simulink model "original"  (R2025a)
settings: Solver=VariableStepAuto  StartTime=0.0  StopTime=800  RelTol=1e-3
undefined symbols (not defined in the file): D1, Delta
libraries: spsThreePhaseSeriesRLCBranchLib x20, spsThreePhaseVIMeasurementLib x18, spsThreePhaseSeriesRLCLoadLib x11, spsRMSLib x8, spsThreePhaseSourceLib x5, spsThreePhaseTransformerTwoWindingsLib x5, spsPMUPLLBasedPositiveSequenceLib x4, spsCurrentMeasurementLib x3, spsPower3phInstantaneousLib x1, spspowerguiLib x1
settings Model: Creator=Subhalaxmi Sahoo  LastModifiedBy=Subhalaxmi Sahoo

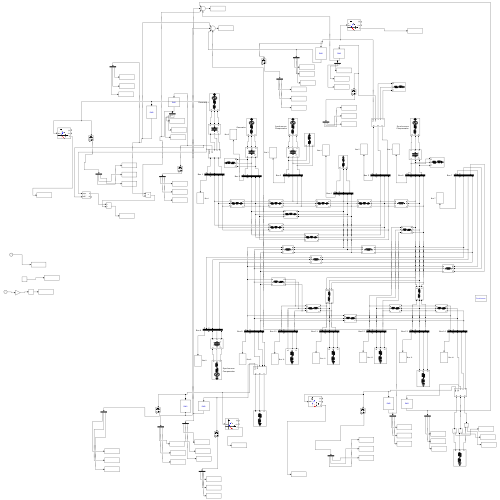
[thumbnail: Simulink's stored preview of the top-level diagram]
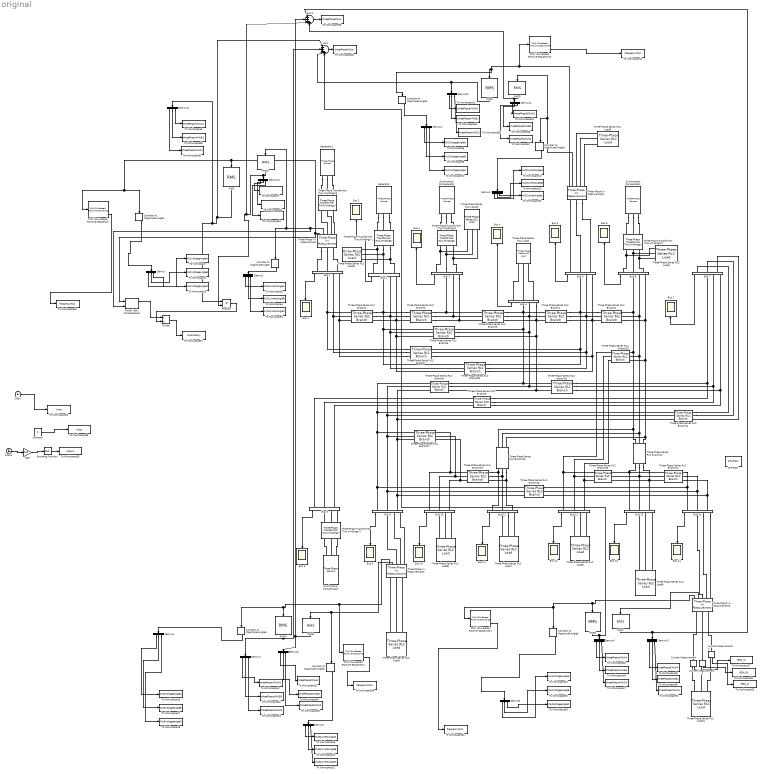
== system original ==
  " Generator" : spsThreePhaseSourceLib/Three-Phase Source  InternalConnection=Yg  VoltagePhases=off  Voltage=1.045  PhaseAngle=-30  Voltage_phases=[25e3 25e3 25e3]/sqrt(3)  PhaseAngles_phases=[0 -120 +120]  Frequency=50  NonIdealSource=on  SpecifyImpedance=on  Resistance=0.8929  Inductance=16.58e-3  ShortCircuitLevel=10  BaseVoltage=1  XRratio=1  BusType=PV  Pref=0.4  Qref=0  Prefabc=[10e3, 10e3, 10e3]  Qrefabc=[0, 0, 0]  Qmin=-0.4  Qmax=0.5
  " Generator1" : spsThreePhaseSourceLib/Three-Phase Source  InternalConnection=Yg  VoltagePhases=off  Voltage=1.06  PhaseAngle=-30  Voltage_phases=[25e3 25e3 25e3]/sqrt(3)  PhaseAngles_phases=[0 -120 +120]  Frequency=50  NonIdealSource=on  SpecifyImpedance=on  Resistance=0.8929  Inductance=16.58e-3  ShortCircuitLevel=10  BaseVoltage=1  XRratio=1  BusType=PQ  Pref=2.324  Qref=-0.169  Prefabc=[10e3, 10e3, 10e3]  Qrefabc=[0, 0, 0]  Qmin=0  Qmax=0
  Bus {1..14} (14 alike) : Scope
      Bus 1 settings: TimeSpan=0.12  ActiveDisplayYMinimum=-1.75  ActiveDisplayYMaximum=1.75
      Bus 10 settings: TimeSpan=0.12  ActiveDisplayYMinimum=-1.5  ActiveDisplayYMaximum=1.5  DataLoggingVariableName=ScopeData9
      Bus 11 settings: TimeSpan=0.12  ActiveDisplayYMinimum=-1.25  ActiveDisplayYMaximum=1.25  DataLoggingVariableName=ScopeData10
      Bus 12 settings: TimeSpan=0.12  ActiveDisplayYMinimum=-1.25  ActiveDisplayYMaximum=1.25  DataLoggingVariableName=ScopeData11
      Bus 13 settings: TimeSpan=0.12  ActiveDisplayYMinimum=-1.25  ActiveDisplayYMaximum=1.25  DataLoggingVariableName=ScopeData12
      Bus 14 settings: TimeSpan=0.12  ActiveDisplayYMinimum=-1.25  ActiveDisplayYMaximum=1.25  DataLoggingVariableName=ScopeData13
      Bus 2 settings: TimeSpan=0.12  ActiveDisplayYMinimum=-1.75  ActiveDisplayYMaximum=1.75
      Bus 3 settings: TimeSpan=0.12  ActiveDisplayYMinimum=-1.75  ActiveDisplayYMaximum=1.75  DataLoggingVariableName=ScopeData6
      Bus 4 settings: TimeSpan=0.12  ActiveDisplayYMinimum=-1.25  ActiveDisplayYMaximum=1.25  DataLoggingVariableName=ScopeData2
      Bus 5 settings: TimeSpan=0.12  ActiveDisplayYMinimum=-1.75  ActiveDisplayYMaximum=2  DataLoggingVariableName=ScopeData3
      Bus 6 settings: TimeSpan=0.12  ActiveDisplayYMinimum=-1.75  ActiveDisplayYMaximum=1.75  DataLoggingVariableName=ScopeData5
      Bus 7 settings: TimeSpan=0.12  ActiveDisplayYMinimum=-1.25  ActiveDisplayYMaximum=1.25  DataLoggingVariableName=ScopeData4
      Bus 8 settings: TimeSpan=0.12  ActiveDisplayYMinimum=-1.1  ActiveDisplayYMaximum=1.1  DataLoggingVariableName=ScopeData7
      Bus 9 settings: TimeSpan=0.12  ActiveDisplayYMinimum=-1  ActiveDisplayYMaximum=0.9  DataLoggingVariableName=ScopeData8
  "Bus 1 " : spsThreePhaseVIMeasurementLib/Three-Phase V-I Measurement  VoltageMeasurement=phase-to-ground  SetLabelV=off  LabelV=Vabc  Vpu=on  VpuLL=off  CurrentMeasurement=yes  SetLabelI=off  LabelI=Iabc  Ipu=on  Pbase=100e6  Vbase=0.95  OutputType=Complex  PhasorSimulation=off  PSBequivalent=0
  "Bus 10 " : spsThreePhaseVIMeasurementLib/Three-Phase V-I Measurement  VoltageMeasurement=phase-to-ground  SetLabelV=off  LabelV=Vabc  Vpu=on  VpuLL=off  CurrentMeasurement=yes  SetLabelI=off  LabelI=Iabc  Ipu=on  Pbase=100e6  Vbase=0.94  OutputType=Complex  PhasorSimulation=off  PSBequivalent=0
  "Bus 11 " : spsThreePhaseVIMeasurementLib/Three-Phase V-I Measurement  VoltageMeasurement=phase-to-ground  SetLabelV=off  LabelV=Vabc  Vpu=on  VpuLL=off  CurrentMeasurement=yes  SetLabelI=off  LabelI=Iabc  Ipu=on  Pbase=100e6  Vbase=0.95  OutputType=Complex  PhasorSimulation=off  PSBequivalent=0
  "Bus 12 " : spsThreePhaseVIMeasurementLib/Three-Phase V-I Measurement  VoltageMeasurement=phase-to-ground  SetLabelV=off  LabelV=Vabc  Vpu=on  VpuLL=off  CurrentMeasurement=yes  SetLabelI=off  LabelI=Iabc  Ipu=on  Pbase=100e6  Vbase=0.95  OutputType=Complex  PhasorSimulation=off  PSBequivalent=0
  "Bus 13 " : spsThreePhaseVIMeasurementLib/Three-Phase V-I Measurement  VoltageMeasurement=phase-to-ground  SetLabelV=off  LabelV=Vabc  Vpu=on  VpuLL=off  CurrentMeasurement=yes  SetLabelI=off  LabelI=Iabc  Ipu=on  Pbase=100e6  Vbase=0.95  OutputType=Complex  PhasorSimulation=off  PSBequivalent=0
  "Bus 14 " : spsThreePhaseVIMeasurementLib/Three-Phase V-I Measurement  VoltageMeasurement=phase-to-ground  SetLabelV=off  LabelV=Vabc  Vpu=on  VpuLL=off  CurrentMeasurement=yes  SetLabelI=off  LabelI=Iabc  Ipu=on  Pbase=100e6  Vbase=0.92  OutputType=Complex  PhasorSimulation=off  PSBequivalent=0
  "Bus 2 " : spsThreePhaseVIMeasurementLib/Three-Phase V-I Measurement  VoltageMeasurement=phase-to-ground  SetLabelV=off  LabelV=Vabc  Vpu=on  VpuLL=off  CurrentMeasurement=yes  SetLabelI=off  LabelI=Iabc  Ipu=on  Pbase=100e6  Vbase=0.95  OutputType=Complex  PhasorSimulation=off  PSBequivalent=0
  "Bus 3 " : spsThreePhaseVIMeasurementLib/Three-Phase V-I Measurement  VoltageMeasurement=phase-to-ground  SetLabelV=off  LabelV=Vabc  Vpu=on  VpuLL=off  CurrentMeasurement=yes  SetLabelI=off  LabelI=Iabc  Ipu=on  Pbase=100e6  Vbase=0.95  OutputType=Complex  PhasorSimulation=off  PSBequivalent=0
  "Bus 4 " : spsThreePhaseVIMeasurementLib/Three-Phase V-I Measurement  VoltageMeasurement=phase-to-ground  SetLabelV=off  LabelV=Vabc  Vpu=on  VpuLL=off  CurrentMeasurement=yes  SetLabelI=off  LabelI=Iabc  Ipu=on  Pbase=100e6  Vbase=0.95  OutputType=Complex  PhasorSimulation=off  PSBequivalent=0
  "Bus 5 " : spsThreePhaseVIMeasurementLib/Three-Phase V-I Measurement  VoltageMeasurement=phase-to-ground  SetLabelV=off  LabelV=Vabc  Vpu=on  VpuLL=off  CurrentMeasurement=yes  SetLabelI=off  LabelI=Iabc  Ipu=on  Pbase=100e6  Vbase=0.95  OutputType=Complex  PhasorSimulation=off  PSBequivalent=0
  "Bus 6 " : spsThreePhaseVIMeasurementLib/Three-Phase V-I Measurement  VoltageMeasurement=phase-to-ground  SetLabelV=off  LabelV=Vabc  Vpu=on  VpuLL=off  CurrentMeasurement=yes  SetLabelI=off  LabelI=Iabc  Ipu=on  Pbase=100e6  Vbase=0.95  OutputType=Complex  PhasorSimulation=off  PSBequivalent=0
  "Bus 7 " : spsThreePhaseVIMeasurementLib/Three-Phase V-I Measurement  VoltageMeasurement=phase-to-ground  SetLabelV=off  LabelV=Vabc  Vpu=on  VpuLL=off  CurrentMeasurement=yes  SetLabelI=off  LabelI=Iabc  Ipu=off  Pbase=100e6  Vbase=0.95  OutputType=Complex  PhasorSimulation=off  PSBequivalent=0
  "Bus 8 " : spsThreePhaseVIMeasurementLib/Three-Phase V-I Measurement  VoltageMeasurement=phase-to-ground  SetLabelV=off  LabelV=Vabc  Vpu=on  VpuLL=off  CurrentMeasurement=yes  SetLabelI=off  LabelI=Iabc  Ipu=on  Pbase=100e6  Vbase=1  OutputType=Complex  PhasorSimulation=off  PSBequivalent=0
  "Bus 9 " : spsThreePhaseVIMeasurementLib/Three-Phase V-I Measurement  VoltageMeasurement=phase-to-ground  SetLabelV=off  LabelV=Vabc  Vpu=on  VpuLL=off  CurrentMeasurement=yes  SetLabelI=off  LabelI=Iabc  Ipu=on  Pbase=100e6  Vbase=0.94  OutputType=Complex  PhasorSimulation=off  PSBequivalent=0
  Clock : Clock
  Clock1 : Clock
  Complex to Magnitude-Angle{,1..6} (7 alike) : ComplexToMagnitudeAngle
  Constant : Constant  Value=0
  Current Measurement : spsCurrentMeasurementLib/Current Measurement  PhasorSimulation=off  OutputType=Complex  PSBequivalent=0
  Current Measurement1 : spsCurrentMeasurementLib/Current Measurement  PhasorSimulation=off  OutputType=Complex  PSBequivalent=0
  Current Measurement2 : spsCurrentMeasurementLib/Current Measurement  PhasorSimulation=off  OutputType=Complex  PSBequivalent=0
  Demux{,1..14} (15 alike) : Demux  Outputs=3
  Divide : Product  Inputs=//
  Gain : Gain  Gain=100
  PMU (PLL-Based, Positive-Sequence){,1..3} (4 alike) : spsPMUPLLBasedPositiveSequenceLib/PMU (PLL-Based, Positive-Sequence)  nominalFrequency=60  samplingRate=64  reportingFactor=1
      settings: LibrarySourceBlock=|
      | sps_lib/Sensors and Measurements/PMU
      | (PLL-Based,
      | Positive-Sequence)
  "Power (3ph, Instantaneous)" : spsPower3phInstantaneousLib/Power (3ph, Instantaneous)
  Product : Product
  RMS{,1..7} (8 alike) : spsRMSLib/RMS  TrueRMS=on  Freq=50  RMSInit=1  Ts=0
  Rounding Function : Rounding
  Sum : Sum  Inputs=|++++
  Sum1 : Sum  Inputs=|++++
  Synchronous Compensator : spsThreePhaseSourceLib/Three-Phase Source  InternalConnection=Yg  VoltagePhases=off  Voltage=1.09  PhaseAngle=-30  Voltage_phases=[25e3 25e3 25e3]/sqrt(3)  PhaseAngles_phases=[0 -120 +120]  Frequency=50  NonIdealSource=on  SpecifyImpedance=on  Resistance=0.8929  Inductance=16.58e-3  ShortCircuitLevel=10  BaseVoltage=1  XRratio=1  BusType=PV  Pref=0  Qref=0  Prefabc=[10e3, 10e3, 10e3]  Qrefabc=[0, 0, 0]  Qmin=-0.06  Qmax=0.24
  Synchronous Compensator : spsThreePhaseSourceLib/Three-Phase Source  InternalConnection=Yg  VoltagePhases=off  Voltage=1.01  PhaseAngle=-30  Voltage_phases=[25e3 25e3 25e3]/sqrt(3)  PhaseAngles_phases=[0 -120 +120]  Frequency=50  NonIdealSource=on  SpecifyImpedance=on  Resistance=0.8929  Inductance=16.58e-3  ShortCircuitLevel=10  BaseVoltage=1  XRratio=1  BusType=PV  Pref=0  Qref=23.4e6  Prefabc=[10e3, 10e3, 10e3]  Qrefabc=[0, 0, 0]  Qmin=0  Qmax=0.4
  "Synchronous Compensator " : spsThreePhaseSourceLib/Three-Phase Source  InternalConnection=Yg  VoltagePhases=off  Voltage=1.07  PhaseAngle=-30  Voltage_phases=[25e3 25e3 25e3]/sqrt(3)  PhaseAngles_phases=[0 -120 +120]  Frequency=50  NonIdealSource=on  SpecifyImpedance=on  Resistance=0.8929  Inductance=16.58e-3  ShortCircuitLevel=10  BaseVoltage=1  XRratio=1  BusType=PV  Pref=0  Qref=23.4e6  Prefabc=[10e3, 10e3, 10e3]  Qrefabc=[0, 0, 0]  Qmin=-0.06  Qmax=0.24
  Three-Phase Series RLC Branch1 : spsThreePhaseSeriesRLCBranchLib/Three-Phase Series RLC Branch  LConnTagsString=A|B|C  RConnTagsString=A|B|C  BranchType=RLC  Resistance=0.01335  Inductance=0.04211/(2*pi*50)  Capacitance=1/0.0128/(2*pi*50)  Measurements=None
  Three-Phase Series RLC Branch10 : spsThreePhaseSeriesRLCBranchLib/Three-Phase Series RLC Branch  LConnTagsString=A|B|C  RConnTagsString=A|B|C  BranchType=L  Resistance=1  Inductance=0.20912/(2*pi*50)  Capacitance=1e-6  Measurements=None
  Three-Phase Series RLC Branch11 : spsThreePhaseSeriesRLCBranchLib/Three-Phase Series RLC Branch  LConnTagsString=A|B|C  RConnTagsString=A|B|C  BranchType=L  Resistance=1  Inductance=0.11001/(2*pi*50)  Capacitance=1e-6  Measurements=None
  Three-Phase Series RLC Branch12 : spsThreePhaseSeriesRLCBranchLib/Three-Phase Series RLC Branch  LConnTagsString=A|B|C  RConnTagsString=A|B|C  BranchType=RL  Resistance=0.06615  Inductance=0.13027/(2*pi*50)  Capacitance=1e-6  Measurements=None
  Three-Phase Series RLC Branch13 : spsThreePhaseSeriesRLCBranchLib/Three-Phase Series RLC Branch  LConnTagsString=A|B|C  RConnTagsString=A|B|C  BranchType=RL  Resistance=0.22092  Inductance=0.19988/(2*pi*50)  Capacitance=1e-6  Measurements=None
  Three-Phase Series RLC Branch14 : spsThreePhaseSeriesRLCBranchLib/Three-Phase Series RLC Branch  LConnTagsString=A|B|C  RConnTagsString=A|B|C  BranchType=RL  Resistance=0.17093  Inductance=0.34802/(2*pi*50)  Capacitance=1e-6  Measurements=None
  Three-Phase Series RLC Branch15 : spsThreePhaseSeriesRLCBranchLib/Three-Phase Series RLC Branch  LConnTagsString=A|B|C  RConnTagsString=A|B|C  BranchType=RL  Resistance=0.12291  Inductance=0.25581/(2*pi*50)  Capacitance=1e-6  Measurements=None
  Three-Phase Series RLC Branch16 : spsThreePhaseSeriesRLCBranchLib/Three-Phase Series RLC Branch  LConnTagsString=A|B|C  RConnTagsString=A|B|C  BranchType=RL  Resistance=0.12711  Inductance=0.27038/(2*pi*50)  Capacitance=1e-6  Measurements=None
  Three-Phase Series RLC Branch17 : spsThreePhaseSeriesRLCBranchLib/Three-Phase Series RLC Branch  LConnTagsString=A|B|C  RConnTagsString=A|B|C  BranchType=RL  Resistance=0.03181  Inductance=0.08450/(2*pi*50)  Capacitance=1e-6  Measurements=None
  Three-Phase Series RLC Branch18 : spsThreePhaseSeriesRLCBranchLib/Three-Phase Series RLC Branch  LConnTagsString=A|B|C  RConnTagsString=A|B|C  BranchType=RL  Resistance=0.09498  Inductance=0.1989/(2*pi*50)  Capacitance=1e-6  Measurements=None
  Three-Phase Series RLC Branch19 : spsThreePhaseSeriesRLCBranchLib/Three-Phase Series RLC Branch  LConnTagsString=A|B|C  RConnTagsString=A|B|C  BranchType=RL  Resistance=0.08205  Inductance=0.19207/(2*pi*50)  Capacitance=1e-6  Measurements=None
  Three-Phase Series RLC Branch2 : spsThreePhaseSeriesRLCBranchLib/Three-Phase Series RLC Branch  LConnTagsString=A|B|C  RConnTagsString=A|B|C  BranchType=RLC  Resistance=0.01938  Inductance=0.05917/(2*pi*50)  Capacitance=1/0.0528/(2*pi*50)  Measurements=None
  Three-Phase Series RLC Branch20 : spsThreePhaseSeriesRLCBranchLib/Three-Phase Series RLC Branch  LConnTagsString=A|B|C  RConnTagsString=A|B|C  BranchType=RLC  Resistance=0.05695  Inductance=0.17388/(2*pi*50)  Capacitance=1/0.0340/(2*pi*50)  Measurements=None
  Three-Phase Series RLC Branch3 : spsThreePhaseSeriesRLCBranchLib/Three-Phase Series RLC Branch  LConnTagsString=A|B|C  RConnTagsString=A|B|C  BranchType=RLC  Resistance=0.04699  Inductance=0.19797/(2*pi*50)  Capacitance=1/0.0438/(2*pi*50)  Measurements=None
  Three-Phase Series RLC Branch4 : spsThreePhaseSeriesRLCBranchLib/Three-Phase Series RLC Branch  LConnTagsString=A|B|C  RConnTagsString=A|B|C  BranchType=L  Resistance=1  Inductance=0.25202/(2*pi*50)  Capacitance=1e-6  Measurements=None
  Three-Phase Series RLC Branch5 : spsThreePhaseSeriesRLCBranchLib/Three-Phase Series RLC Branch  LConnTagsString=A|B|C  RConnTagsString=A|B|C  BranchType=RLC  Resistance=0.06701  Inductance=0.17103/(2*pi*50)  Capacitance=1/0.0346/(2*pi*50)  Measurements=None
  Three-Phase Series RLC Branch6 : spsThreePhaseSeriesRLCBranchLib/Three-Phase Series RLC Branch  LConnTagsString=A|B|C  RConnTagsString=A|B|C  BranchType=RLC  Resistance=0.05811  Inductance=0.17632/(2*pi*50)  Capacitance=1/0.0374/(2*pi*50)  Measurements=None
  Three-Phase Series RLC Branch7 : spsThreePhaseSeriesRLCBranchLib/Three-Phase Series RLC Branch  LConnTagsString=A|B|C  RConnTagsString=A|B|C  BranchType=RLC  Resistance=0.05403  Inductance=0.22304/(2*pi*50)  Capacitance=1/0.0492/(2*pi*50)  Measurements=None
  Three-Phase Series RLC Branch8 : spsThreePhaseSeriesRLCBranchLib/Three-Phase Series RLC Branch  LConnTagsString=A|B|C  RConnTagsString=A|B|C  BranchType=L  Resistance=1  Inductance=0.55618/(2*pi*50)  Capacitance=1e-6  Measurements=None
  Three-Phase Series RLC Branch9 : spsThreePhaseSeriesRLCBranchLib/Three-Phase Series RLC Branch  LConnTagsString=A|B|C  RConnTagsString=A|B|C  BranchType=L  Resistance=1  Inductance=0.17615/(2*pi*50)  Capacitance=1e-6  Measurements=None
  Three-Phase Series RLC Load1 : spsThreePhaseSeriesRLCLoadLib/Three-Phase Series RLC Load  LConnTagsString=A|B|C  Configuration=Y (grounded)  NominalVoltage=1  Vabc=[1e3 1e3 1e3]  Vabcp=[1e3 1e3 1e3]  NominalFrequency=50  UnbalancedPower=off  ActivePower=0.478  InductivePower=0  CapacitivePower=0.039  Pabc=[10e3 9e3 11e3]  QLabc=[100 90 110]  QCabc=[100 90 110]  Pabcp=[10e3 9e3 11e3]  QLabcp=[100 90 110]  QCabcp=[100 90 110]  Measurements=None  LoadType=constant PQ
  Three-Phase Series RLC Load10 : spsThreePhaseSeriesRLCLoadLib/Three-Phase Series RLC Load  LConnTagsString=A|B|C  Configuration=Y (grounded)  NominalVoltage=1  Vabc=[1e3 1e3 1e3]  Vabcp=[1e3 1e3 1e3]  NominalFrequency=50  UnbalancedPower=off  ActivePower=0.149  InductivePower=0.050  CapacitivePower=0  Pabc=[10e3 9e3 11e3]  QLabc=[100 90 110]  QCabc=[100 90 110]  Pabcp=[10e3 9e3 11e3]  QLabcp=[100 90 110]  QCabcp=[100 90 110]  Measurements=None  LoadType=constant Z
  Three-Phase Series RLC Load11 : spsThreePhaseSeriesRLCLoadLib/Three-Phase Series RLC Load  LConnTagsString=A|B|C  Configuration=Y (grounded)  NominalVoltage=1  Vabc=[1e3 1e3 1e3]  Vabcp=[1e3 1e3 1e3]  NominalFrequency=50  UnbalancedPower=off  ActivePower=0.217  InductivePower=0.127  CapacitivePower=0  Pabc=[10e3 9e3 11e3]  QLabc=[100 90 110]  QCabc=[100 90 110]  Pabcp=[10e3 9e3 11e3]  QLabcp=[100 90 110]  QCabcp=[100 90 110]  Measurements=None  LoadType=constant PQ
  Three-Phase Series RLC Load12 : spsThreePhaseSeriesRLCLoadLib/Three-Phase Series RLC Load  LConnTagsString=A|B|C  Configuration=Y (grounded)  NominalVoltage=1  Vabc=[1e3 1e3 1e3]  Vabcp=[1e3 1e3 1e3]  NominalFrequency=50  UnbalancedPower=off  ActivePower=0.942  InductivePower=0.191  CapacitivePower=0  Pabc=[10e3 9e3 11e3]  QLabc=[100 90 110]  QCabc=[100 90 110]  Pabcp=[10e3 9e3 11e3]  QLabcp=[100 90 110]  QCabcp=[100 90 110]  Measurements=None  LoadType=constant PQ
  Three-Phase Series RLC Load3 : spsThreePhaseSeriesRLCLoadLib/Three-Phase Series RLC Load  LConnTagsString=A|B|C  Configuration=Y (grounded)  NominalVoltage=1  Vabc=[1e3 1e3 1e3]  Vabcp=[1e3 1e3 1e3]  NominalFrequency=50  UnbalancedPower=off  ActivePower=0.076  InductivePower=0.016  CapacitivePower=0  Pabc=[10e3 9e3 11e3]  QLabc=[100 90 110]  QCabc=[100 90 110]  Pabcp=[10e3 9e3 11e3]  QLabcp=[100 90 110]  QCabcp=[100 90 110]  Measurements=None  LoadType=constant PQ
  Three-Phase Series RLC Load4 : spsThreePhaseSeriesRLCLoadLib/Three-Phase Series RLC Load  LConnTagsString=A|B|C  Configuration=Y (grounded)  NominalVoltage=1  Vabc=[1e3 1e3 1e3]  Vabcp=[1e3 1e3 1e3]  NominalFrequency=50  UnbalancedPower=off  ActivePower=0.112  InductivePower=0.075  CapacitivePower=0  Pabc=[10e3 9e3 11e3]  QLabc=[100 90 110]  QCabc=[100 90 110]  Pabcp=[10e3 9e3 11e3]  QLabcp=[100 90 110]  QCabcp=[100 90 110]  Measurements=None  LoadType=constant PQ
  Three-Phase Series RLC Load5 : spsThreePhaseSeriesRLCLoadLib/Three-Phase Series RLC Load  LConnTagsString=A|B|C  Configuration=Y (grounded)  NominalVoltage=1  Vabc=[1e3 1e3 1e3]  Vabcp=[1e3 1e3 1e3]  NominalFrequency=50  UnbalancedPower=off  ActivePower=0.295  InductivePower=0.166  CapacitivePower=0  Pabc=[10e3 9e3 11e3]  QLabc=[100 90 110]  QCabc=[100 90 110]  Pabcp=[10e3 9e3 11e3]  QLabcp=[100 90 110]  QCabcp=[100 90 110]  Measurements=None  LoadType=constant PQ
  Three-Phase Series RLC Load6 : spsThreePhaseSeriesRLCLoadLib/Three-Phase Series RLC Load  LConnTagsString=A|B|C  Configuration=Y (grounded)  NominalVoltage=1  Vabc=[1e3 1e3 1e3]  Vabcp=[1e3 1e3 1e3]  NominalFrequency=50  UnbalancedPower=off  ActivePower=0.09  InductivePower=0.058  CapacitivePower=0  Pabc=[10e3 9e3 11e3]  QLabc=[100 90 110]  QCabc=[100 90 110]  Pabcp=[10e3 9e3 11e3]  QLabcp=[100 90 110]  QCabcp=[100 90 110]  Measurements=None  LoadType=constant PQ
  Three-Phase Series RLC Load7 : spsThreePhaseSeriesRLCLoadLib/Three-Phase Series RLC Load  LConnTagsString=A|B|C  Configuration=Y (grounded)  NominalVoltage=1  Vabc=[1e3 1e3 1e3]  Vabcp=[1e3 1e3 1e3]  NominalFrequency=50  UnbalancedPower=off  ActivePower=0.035  InductivePower=0.018  CapacitivePower=0  Pabc=[10e3 9e3 11e3]  QLabc=[100 90 110]  QCabc=[100 90 110]  Pabcp=[10e3 9e3 11e3]  QLabcp=[100 90 110]  QCabcp=[100 90 110]  Measurements=None  LoadType=constant PQ
  Three-Phase Series RLC Load8 : spsThreePhaseSeriesRLCLoadLib/Three-Phase Series RLC Load  LConnTagsString=A|B|C  Configuration=Y (grounded)  NominalVoltage=1  Vabc=[1e3 1e3 1e3]  Vabcp=[1e3 1e3 1e3]  NominalFrequency=50  UnbalancedPower=off  ActivePower=0.061  InductivePower=0.016  CapacitivePower=0  Pabc=[10e3 9e3 11e3]  QLabc=[100 90 110]  QCabc=[100 90 110]  Pabcp=[10e3 9e3 11e3]  QLabcp=[100 90 110]  QCabcp=[100 90 110]  Measurements=None  LoadType=constant PQ
  Three-Phase Series RLC Load9 : spsThreePhaseSeriesRLCLoadLib/Three-Phase Series RLC Load  LConnTagsString=A|B|C  Configuration=Y (grounded)  NominalVoltage=1  Vabc=[1e3 1e3 1e3]  Vabcp=[1e3 1e3 1e3]  NominalFrequency=50  UnbalancedPower=off  ActivePower=0.135  InductivePower=0.058  CapacitivePower=0  Pabc=[10e3 9e3 11e3]  QLabc=[100 90 110]  QCabc=[100 90 110]  Pabcp=[10e3 9e3 11e3]  QLabcp=[100 90 110]  QCabcp=[100 90 110]  Measurements=None  LoadType=constant PQ
  Three-Phase Transformer (Two Windings)1 : spsThreePhaseTransformerTwoWindingsLib/Three-Phase Transformer (Two Windings)  Winding1Connection=Delta (D1)  Winding2Connection=Yg  CoreType=Three single-phase transformers  SetSaturation=off  Hysteresis=off  DataFile='hysteresis'  SetInitialFlux=off  Measurements=None  UNITS=pu  NominalPower=[ 1 , 50 ]  Winding1=[ 1.045 , 0.002 , 0.08 ]  Winding2=[ 1.045 , 0.002 , 0.08 ]  Rm=500  Lm=500  L0=0.5  Saturation=[ 0,0 ; 0.0024,1.2 ; 1.0,1.52 ]  InitialFluxes=[ 0.8 , -0.8 , 0.7 ]  BreakLoop=off  DiscreteSolver=Trapezoidal iterative  DataType=off  TransfoNumber=1
  Three-Phase Transformer (Two Windings)2 : spsThreePhaseTransformerTwoWindingsLib/Three-Phase Transformer (Two Windings)  Winding1Connection=Delta (D1)  Winding2Connection=Yg  CoreType=Three single-phase transformers  SetSaturation=off  Hysteresis=off  DataFile='hysteresis'  SetInitialFlux=off  Measurements=None  UNITS=pu  NominalPower=[ 1 , 50 ]  Winding1=[ 1.01 , 0.002 , 0.08 ]  Winding2=[ 1.01 , 0.002 , 0.08 ]  Rm=500  Lm=500  L0=0.5  Saturation=[ 0,0 ; 0.0024,1.2 ; 1.0,1.52 ]  InitialFluxes=[ 0.8 , -0.8 , 0.7 ]  BreakLoop=off  DiscreteSolver=Trapezoidal iterative  DataType=off  TransfoNumber=1
  Three-Phase Transformer (Two Windings)3 : spsThreePhaseTransformerTwoWindingsLib/Three-Phase Transformer (Two Windings)  Winding1Connection=Delta (D1)  Winding2Connection=Yg  CoreType=Three single-phase transformers  SetSaturation=off  Hysteresis=off  DataFile='hysteresis'  SetInitialFlux=off  Measurements=None  UNITS=pu  NominalPower=[ 1 , 50 ]  Winding1=[ 1.07 , 0.002 , 0.08 ]  Winding2=[ 1.07 , 0.002 , 0.08 ]  Rm=500  Lm=500  L0=0.5  Saturation=[ 0,0 ; 0.0024,1.2 ; 1.0,1.52 ]  InitialFluxes=[ 0.8 , -0.8 , 0.7 ]  BreakLoop=off  DiscreteSolver=Trapezoidal iterative  DataType=off  TransfoNumber=1
  Three-Phase Transformer (Two Windings)4 : spsThreePhaseTransformerTwoWindingsLib/Three-Phase Transformer (Two Windings)  Winding1Connection=Yg  Winding2Connection=Delta (D1)  CoreType=Three single-phase transformers  SetSaturation=off  Hysteresis=off  DataFile='hysteresis'  SetInitialFlux=off  Measurements=None  UNITS=pu  NominalPower=[ 1 , 50 ]  Winding1=[ 1.09 , 0.002 , 0.08]  Winding2=[1.09 , 0.002 , 0.08]  Rm=500  Lm=500  L0=0.5  Saturation=[0 0;0.0023999 1.2;1 1.52]  InitialFluxes=[0.80002 -0.80002 0.69999]  BreakLoop=off  DiscreteSolver=Trapezoidal iterative  DataType=off  TransfoNumber=1
  Three-Phase Transformer (Two Windings)5 : spsThreePhaseTransformerTwoWindingsLib/Three-Phase Transformer (Two Windings)  Winding1Connection=Delta (D1)  Winding2Connection=Yg  CoreType=Three single-phase transformers  SetSaturation=off  Hysteresis=off  DataFile='hysteresis'  SetInitialFlux=off  Measurements=None  UNITS=pu  NominalPower=[ 1 , 50 ]  Winding1=[ 1.06 , 0.002 , 0.08 ]  Winding2=[ 1.06 , 0.002 , 0.08 ]  Rm=500  Lm=500  L0=0.5  Saturation=[ 0,0 ; 0.0024,1.2 ; 1.0,1.52 ]  InitialFluxes=[ 0.8 , -0.8 , 0.7 ]  BreakLoop=off  DiscreteSolver=Trapezoidal iterative  DataType=off  TransfoNumber=1
  Three-Phase V-I Measurement{,1..3} (4 alike) : spsThreePhaseVIMeasurementLib/Three-Phase V-I Measurement  VoltageMeasurement=phase-to-ground  SetLabelV=off  LabelV=Vabc  Vpu=off  VpuLL=off  CurrentMeasurement=yes  SetLabelI=off  LabelI=Iabc  Ipu=off  Pbase=100e6  Vbase=500e3  OutputType=Complex  PhasorSimulation=off  PSBequivalent=0
  To Workspace : ToWorkspace  VariableName=MU1VoltageAngleA  SampleTime=0.2
      settings: Save2DSignal=2-D array (concatenate along first dimension)
  To Workspace1 : ToWorkspace  VariableName=MU1VoltageAngleB  SampleTime=0.2
      settings: Save2DSignal=2-D array (concatenate along first dimension)
  To Workspace10 : ToWorkspace  VariableName=MU2VoltageAngleC  SampleTime=0.2
      settings: Save2DSignal=2-D array (concatenate along first dimension)
  To Workspace11 : ToWorkspace  VariableName=MU2CurrentAngleA  SampleTime=0.2
      settings: Save2DSignal=2-D array (concatenate along first dimension)
  To Workspace12 : ToWorkspace  VariableName=MU2CurrentAngleB  SampleTime=0.2
      settings: Save2DSignal=2-D array (concatenate along first dimension)
  To Workspace13 : ToWorkspace  VariableName=MU2CurrentAngleC  SampleTime=0.2
      settings: Save2DSignal=2-D array (concatenate along first dimension)
  To Workspace14 : ToWorkspace  VariableName=threePhaseVMUA2  SampleTime=0.2
      settings: Save2DSignal=2-D array (concatenate along first dimension)
  To Workspace15 : ToWorkspace  VariableName=threePhaseCMUA2  SampleTime=0.2
      settings: Save2DSignal=2-D array (concatenate along first dimension)
  To Workspace16 : ToWorkspace  VariableName=MU3VoltageAngleA  SampleTime=0.2
      settings: Save2DSignal=2-D array (concatenate along first dimension)
  To Workspace17 : ToWorkspace  VariableName=MU3VoltageAngleB  SampleTime=0.2
      settings: Save2DSignal=2-D array (concatenate along first dimension)
  To Workspace18 : ToWorkspace  VariableName=MU3VoltageAngleC  SampleTime=0.2
      settings: Save2DSignal=2-D array (concatenate along first dimension)
  To Workspace19 : ToWorkspace  VariableName=MU3CurrentAngleA  SampleTime=0.2
      settings: Save2DSignal=2-D array (concatenate along first dimension)
  To Workspace2 : ToWorkspace  VariableName=MU1VoltageAngleC  SampleTime=0.2
      settings: Save2DSignal=2-D array (concatenate along first dimension)
  To Workspace20 : ToWorkspace  VariableName=MU3CurrentAngleB  SampleTime=0.2
      settings: Save2DSignal=2-D array (concatenate along first dimension)
  To Workspace21 : ToWorkspace  VariableName=MU3CurrentAngleC  SampleTime=0.2
      settings: Save2DSignal=2-D array (concatenate along first dimension)
  To Workspace22 : ToWorkspace  VariableName=threePhaseVMUB3  SampleTime=0.2
      settings: Save2DSignal=2-D array (concatenate along first dimension)
  To Workspace23 : ToWorkspace  VariableName=threePhaseCMUA3  SampleTime=0.2
      settings: Save2DSignal=2-D array (concatenate along first dimension)
  To Workspace24 : ToWorkspace  VariableName=MU4VoltageAngleA  SampleTime=0.2
      settings: Save2DSignal=2-D array (concatenate along first dimension)
  To Workspace25 : ToWorkspace  VariableName=MU4VoltageAngleB  SampleTime=0.2
      settings: Save2DSignal=2-D array (concatenate along first dimension)
  To Workspace26 : ToWorkspace  VariableName=MU4VoltageAngleC  SampleTime=0.2
      settings: Save2DSignal=2-D array (concatenate along first dimension)
  To Workspace27 : ToWorkspace  VariableName=IED4_iA  SampleTime=0.2
      settings: Save2DSignal=2-D array (concatenate along first dimension)
  To Workspace28 : ToWorkspace  VariableName=IED4_iB  SampleTime=0.2
      settings: Save2DSignal=2-D array (concatenate along first dimension)
  To Workspace29 : ToWorkspace  VariableName=IED4_iC  SampleTime=0.2
      settings: Save2DSignal=2-D array (concatenate along first dimension)
  To Workspace3 : ToWorkspace  VariableName=MU1CurrentAngleA  SampleTime=0.2
      settings: Save2DSignal=2-D array (concatenate along first dimension)
  To Workspace30 : ToWorkspace  VariableName=threePhaseVMUA4  SampleTime=0.2
      settings: Save2DSignal=2-D array (concatenate along first dimension)
  To Workspace31 : ToWorkspace  VariableName=threePhaseCMUC4  SampleTime=0.2
      settings: Save2DSignal=2-D array (concatenate along first dimension)
  To Workspace32 : ToWorkspace  VariableName=time  SampleTime=0.2
      settings: Save2DSignal=2-D array (concatenate along first dimension)
  To Workspace33 : ToWorkspace  VariableName=sqNum  SampleTime=0.2
      settings: Save2DSignal=2-D array (concatenate along first dimension)
  To Workspace34 : ToWorkspace  VariableName=frequencyMU1  SampleTime=0.2
      settings: Save2DSignal=2-D array (concatenate along first dimension)
  To Workspace35 : ToWorkspace  VariableName=threePhaseVSum  SampleTime=0.2
      settings: Save2DSignal=2-D array (concatenate along first dimension)
  To Workspace36 : ToWorkspace  VariableName=threePhaseCSum  SampleTime=0.2
      settings: Save2DSignal=2-D array (concatenate along first dimension)
  To Workspace37 : ToWorkspace  VariableName=consistency  SampleTime=0.2
      settings: Save2DSignal=2-D array (concatenate along first dimension)
  To Workspace38 : ToWorkspace  VariableName=class  SampleTime=0.2
      settings: Save2DSignal=2-D array (concatenate along first dimension)
  To Workspace39 : ToWorkspace  VariableName=frequencyMU3  SampleTime=0.2
      settings: Save2DSignal=2-D array (concatenate along first dimension)
  To Workspace4 : ToWorkspace  VariableName=MU1CurrentAngleB  SampleTime=0.2
      settings: Save2DSignal=2-D array (concatenate along first dimension)
  To Workspace40 : ToWorkspace  VariableName=frequencyMU4  SampleTime=0.2
      settings: Save2DSignal=2-D array (concatenate along first dimension)
  To Workspace41 : ToWorkspace  VariableName=frequencyMU2  SampleTime=0.2
      settings: Save2DSignal=2-D array (concatenate along first dimension)
  To Workspace42 : ToWorkspace  VariableName=threePhaseVMUA3  SampleTime=0.2
      settings: Save2DSignal=2-D array (concatenate along first dimension)
  To Workspace43 : ToWorkspace  VariableName=threePhaseVMUC3  SampleTime=0.2
      settings: Save2DSignal=2-D array (concatenate along first dimension)
  To Workspace44 : ToWorkspace  VariableName=threePhaseCMUB3  SampleTime=0.2
      settings: Save2DSignal=2-D array (concatenate along first dimension)
  To Workspace45 : ToWorkspace  VariableName=threePhaseCMUC3  SampleTime=0.2
      settings: Save2DSignal=2-D array (concatenate along first dimension)
  To Workspace46 : ToWorkspace  VariableName=threePhaseVMUB4  SampleTime=0.2
      settings: Save2DSignal=2-D array (concatenate along first dimension)
  To Workspace47 : ToWorkspace  VariableName=threePhaseVMUC4  SampleTime=0.2
      settings: Save2DSignal=2-D array (concatenate along first dimension)
  To Workspace48 : ToWorkspace  VariableName=threePhaseCMUB4  SampleTime=0.2
      settings: Save2DSignal=2-D array (concatenate along first dimension)
  To Workspace49 : ToWorkspace  VariableName=threePhaseCMUA4  SampleTime=0.2
      settings: Save2DSignal=2-D array (concatenate along first dimension)
  To Workspace5 : ToWorkspace  VariableName=MU1CurrentAngleC  SampleTime=0.2
      settings: Save2DSignal=2-D array (concatenate along first dimension)
  To Workspace50 : ToWorkspace  VariableName=threePhaseVMUB1  SampleTime=0.2
      settings: Save2DSignal=2-D array (concatenate along first dimension)
  To Workspace51 : ToWorkspace  VariableName=threePhaseVMUC1  SampleTime=0.2
      settings: Save2DSignal=2-D array (concatenate along first dimension)
  To Workspace52 : ToWorkspace  VariableName=threePhaseCurrentMUB1  SampleTime=0.2
      settings: Save2DSignal=2-D array (concatenate along first dimension)
  To Workspace53 : ToWorkspace  VariableName=threePhaseCurrentMUC1  SampleTime=0.2
      settings: Save2DSignal=2-D array (concatenate along first dimension)
  To Workspace54 : ToWorkspace  VariableName=threePhaseVMUB2  SampleTime=0.2
      settings: Save2DSignal=2-D array (concatenate along first dimension)
  To Workspace55 : ToWorkspace  VariableName=threePhaseVMUC2  SampleTime=0.2
      settings: Save2DSignal=2-D array (concatenate along first dimension)
  To Workspace56 : ToWorkspace  VariableName=threePhaseCMUB2  SampleTime=0.2
      settings: Save2DSignal=2-D array (concatenate along first dimension)
  To Workspace57 : ToWorkspace  VariableName=threePhaseCMUC2  SampleTime=0.2
      settings: Save2DSignal=2-D array (concatenate along first dimension)
  To Workspace6 : ToWorkspace  VariableName=threePhaseVMUA1  SampleTime=0.2
      settings: Save2DSignal=2-D array (concatenate along first dimension)
  To Workspace7 : ToWorkspace  VariableName=threePhaseCurrentMUA1  SampleTime=0.2
      settings: Save2DSignal=2-D array (concatenate along first dimension)
  To Workspace8 : ToWorkspace  VariableName=MU2VoltageAngleA  SampleTime=0.2
      settings: Save2DSignal=2-D array (concatenate along first dimension)
  To Workspace9 : ToWorkspace  VariableName=MU2VoltageAngleB  SampleTime=0.2
      settings: Save2DSignal=2-D array (concatenate along first dimension)
  powergui : spspowerguiLib/powergui  Priority=1  SimulationMode=Continuous  SampleTime=50e-6  frequency=60  Iterations=50  frequencyindice=50  Pbase=100e6  ErrMax=1e-4  UnitsV=kV  UnitsW=MW  buscounter=0  FunctionMessages=off  echomessages=off  EnableUseOfTLC=off  CurrentSourceSwitches=on  DisableSnubberDevices=off  DisableRonSwitches=off  DisableVfSwitches=off  DisplayEquations=off  AutomaticDiscreteSolvers=off  SolverType=Tustin  Interpol=off  ExternalGateDelay=off  methode=off  Ts=100  x0status=blocks  SPID=off  SwTol=0  HookPort=off  NonlinearTolerance=1e-4  nMaxIteration=100  ContinueOnMaxIteration=off  RestoreLinks=warning  ResistiveCurrentMeasurement=off  Frange=[0:2:500]  Ylog=off  Xlog=on  ShowGrid=off  save=off  variable=ZData  structure=0  ZoomFFT=off  StartTime=0.0  cycles=1  DisplayStyle=1  fundamental=60  FreqAxis=off  MaxFrequency=1000  frequencyindicesteady=1  RmsSteady=1  display=off
  wires:
  RMS7/1 -> Demux10/1, Sum1/1
  Demux5/2 -> To Workspace20/1
  Demux10/3 -> To Workspace31/1
  Demux3/1 -> To Workspace11/1
  "Power (3ph, Instantaneous)"/1 -> Divide/1
  Clock1/1 -> Gain/1
  "Bus 11 "/1 -> Bus 11/1
  Demux4/3 -> To Workspace18/1
  Demux6/2 -> To Workspace25/1
  "Bus 10 "/1 -> Bus 10/1
  "Bus 13 "/1 -> Bus 13/1
  Demux/3 -> To Workspace2/1
  Complex to Magnitude-Angle/2 -> Demux1/1
  Sum/1 -> To Workspace35/1
  Demux10/2 -> To Workspace48/1
  Three-Phase V-I Measurement2/1 -> "PMU (PLL-Based, Positive-Sequence)1"/1, Complex to Magnitude-Angle4/1, RMS4/1
  Three-Phase V-I Measurement3/2 -> RMS7/1
  Demux11/3 -> To Workspace6/1
  RMS2/1 -> Sum/3, Demux13/1
  Clock/1 -> To Workspace32/1
  Current Measurement/1 -> To Workspace27/1
  RMS3/1 -> Demux14/1, Sum1/4
  Demux1/3 -> To Workspace5/1
  Demux7/3 -> To Workspace43/1
  "Bus 5 "/1 -> Bus 5/1
  Complex to Magnitude-Angle3/2 -> Demux3/1
  Three-Phase V-I Measurement1/1 -> "PMU (PLL-Based, Positive-Sequence)3"/1, Complex to Magnitude-Angle2/1, RMS2/1
  Demux14/3 -> To Workspace57/1
  Demux14/1 -> To Workspace15/1
  "Bus 9 "/1 -> Bus 9/1
  Complex to Magnitude-Angle6/2 -> Demux6/1
  Demux1/1 -> To Workspace3/1
  Demux4/1 -> To Workspace16/1
  "PMU (PLL-Based, Positive-Sequence)"/3 -> To Workspace34/1
  "Bus 12 "/1 -> Bus 12/1
  Demux3/3 -> To Workspace13/1
  Demux5/1 -> To Workspace19/1
  Gain/1 -> Rounding Function/1
  "Bus 2 "/1 -> Bus 2/1
  "Bus 6 "/1 -> Bus 6/1
  Demux13/1 -> To Workspace14/1
  Complex to Magnitude-Angle5/2 -> Demux5/1
  Complex to Magnitude-Angle4/2 -> Demux4/1
  Demux/1 -> To Workspace/1
  Three-Phase V-I Measurement1/2 -> Complex to Magnitude-Angle3/1, RMS3/1
  Demux7/2 -> To Workspace22/1
  Demux11/1 -> To Workspace51/1
  Complex to Magnitude-Angle1/2 -> Demux/1
  "Bus 14 "/1 -> Bus 14/1
  Demux2/2 -> To Workspace9/1
  Product/1 -> Divide/2
  Demux13/2 -> To Workspace54/1
  Current Measurement1/1 -> To Workspace28/1
  Rounding Function/1 -> To Workspace33/1
  Sum1/1 -> To Workspace36/1
  Complex to Magnitude-Angle2/2 -> Demux2/1
  Demux3/2 -> To Workspace12/1
  Three-Phase V-I Measurement/2 -> "Power (3ph, Instantaneous)"/2, Complex to Magnitude-Angle/1, RMS1/1
  Demux11/2 -> To Workspace50/1
  Demux10/1 -> To Workspace49/1
  Demux/2 -> To Workspace1/1
  Demux2/3 -> To Workspace10/1
  Constant/1 -> To Workspace38/1
  Demux14/2 -> To Workspace56/1
  RMS4/1 -> Demux7/1, Sum/2
  "Bus 7 "/1 -> Bus 7/1
  "PMU (PLL-Based, Positive-Sequence)3"/3 -> To Workspace41/1
  Demux2/1 -> To Workspace8/1
  Demux1/2 -> To Workspace4/1
  "PMU (PLL-Based, Positive-Sequence)1"/3 -> To Workspace39/1
  Demux9/3 -> To Workspace47/1
  Three-Phase V-I Measurement/1 -> RMS/1, Complex to Magnitude-Angle1/1, "PMU (PLL-Based, Positive-Sequence)"/1, "Power (3ph, Instantaneous)"/1
  Demux12/1 -> To Workspace7/1
  Demux6/3 -> To Workspace26/1
  Three-Phase V-I Measurement2/2 -> Complex to Magnitude-Angle5/1, RMS5/1
  Demux5/3 -> To Workspace21/1
  "Bus 3 "/1 -> Bus 3/1
  Demux6/1 -> To Workspace24/1
  RMS5/1 -> Demux8/1, Sum1/2
  Demux9/2 -> To Workspace46/1
  Demux8/3 -> To Workspace45/1
  "Bus 8 "/1 -> Bus 8/1
  Demux8/1 -> To Workspace23/1
  Demux7/1 -> To Workspace42/1
  "Bus 4 "/1 -> Bus 4/1
  RMS/1 -> Product/1, Demux11/1, Sum/1
  Demux4/2 -> To Workspace17/1
  "PMU (PLL-Based, Positive-Sequence)2"/3 -> To Workspace40/1
  Current Measurement2/1 -> To Workspace29/1
  Divide/1 -> To Workspace37/1
  Demux8/2 -> To Workspace44/1
  Three-Phase V-I Measurement3/1 -> "PMU (PLL-Based, Positive-Sequence)2"/1, Complex to Magnitude-Angle6/1, RMS6/1
  Demux13/3 -> To Workspace55/1
  Demux12/2 -> To Workspace52/1
  Demux9/1 -> To Workspace30/1
  "Bus 1 "/1 -> Bus 1/1
  RMS6/1 -> Demux9/1, Sum/4
  RMS1/1 -> Demux12/1, Sum1/3, Product/2
  Demux12/3 -> To Workspace53/1
  connections:
  Three-Phase Series RLC Branch7/LConn3 -- "Bus 1 "/RConn3 -- Three-Phase Series RLC Branch2/LConn3
  Three-Phase Series RLC Branch3/RConn2 -- "Bus 3 "/RConn2 -- Three-Phase Series RLC Branch5/LConn2
  Three-Phase Series RLC Branch7/LConn2 -- "Bus 1 "/RConn2 -- Three-Phase Series RLC Branch2/LConn2
  Three-Phase Transformer (Two Windings)3/RConn3 -- "Bus 6 "/LConn3 -- Three-Phase Series RLC Load4/LConn3
  Three-Phase Series RLC Branch3/LConn1 -- "Bus 2 "/RConn1 -- Three-Phase Series RLC Branch20/LConn1 -- Three-Phase Series RLC Branch6/LConn1 -- Three-Phase Series RLC Branch2/RConn1
  Three-Phase Series RLC Branch8/RConn1 -- "Bus 4 "/RConn1 -- Three-Phase Series RLC Branch1/LConn1 -- Three-Phase Series RLC Branch5/RConn1 -- Three-Phase Series RLC Branch6/RConn1 -- Three-Phase Series RLC Branch10/LConn1
  Three-Phase Series RLC Branch8/RConn3 -- "Bus 4 "/RConn3 -- Three-Phase Series RLC Branch1/LConn3 -- Three-Phase Series RLC Branch5/RConn3 -- Three-Phase Series RLC Branch6/RConn3 -- Three-Phase Series RLC Branch10/LConn3
  Three-Phase Series RLC Branch15/RConn1 -- "Bus 12 "/LConn1 -- Three-Phase Series RLC Branch13/RConn1
  Three-Phase Series RLC Branch13/LConn2 -- "Bus 13 "/LConn2 -- Three-Phase Series RLC Branch14/RConn2 -- Three-Phase Series RLC Branch12/RConn2
  Three-Phase Series RLC Branch9/RConn1 -- "Bus 7 "/RConn1 -- Three-Phase Series RLC Branch10/RConn1
  Three-Phase Series RLC Branch14/LConn1 -- "Bus 14 "/LConn1 -- Three-Phase Series RLC Branch16/LConn1
  Three-Phase Series RLC Branch7/LConn1 -- "Bus 1 "/RConn1 -- Three-Phase Series RLC Branch2/LConn1
  Three-Phase Transformer (Two Windings)3/RConn2 -- "Bus 6 "/LConn2 -- Three-Phase Series RLC Load4/LConn2
  Three-Phase Series RLC Branch13/LConn1 -- "Bus 13 "/LConn1 -- Three-Phase Series RLC Branch14/RConn1 -- Three-Phase Series RLC Branch12/RConn1
  "Bus 3 "/LConn2 -- Three-Phase Series RLC Load12/LConn2 -- Three-Phase Transformer (Two Windings)2/RConn2
  Three-Phase Series RLC Branch2/RConn3 -- "Bus 2 "/RConn3 -- Three-Phase Series RLC Branch20/LConn3 -- Three-Phase Series RLC Branch6/LConn3 -- Three-Phase Series RLC Branch3/LConn3
  Three-Phase Series RLC Branch14/LConn2 -- "Bus 14 "/LConn2 -- Three-Phase Series RLC Branch16/LConn2
  Three-Phase Transformer (Two Windings)1/RConn2 -- "Bus 2 "/LConn2 -- Three-Phase Series RLC Load11/LConn2
  Three-Phase Series RLC Branch9/RConn2 -- "Bus 7 "/RConn2 -- Three-Phase Series RLC Branch10/RConn2
  Three-Phase Series RLC Branch15/RConn3 -- "Bus 12 "/LConn3 -- Three-Phase Series RLC Branch13/RConn3
  Three-Phase Series RLC Branch3/RConn1 -- "Bus 3 "/RConn1 -- Three-Phase Series RLC Branch5/LConn1
  Three-Phase Series RLC Branch8/LConn2 -- Three-Phase Series RLC Branch11/RConn2 -- "Bus 9 "/LConn2 -- Three-Phase Series RLC Branch16/RConn2 -- Three-Phase Series RLC Branch17/RConn2
  Three-Phase Series RLC Branch18/RConn1 -- "Bus 11 "/LConn1 -- Three-Phase Series RLC Branch19/RConn1
  Three-Phase Series RLC Branch19/LConn3 -- "Bus 10 "/LConn3 -- Three-Phase Series RLC Branch17/LConn3
  Three-Phase Series RLC Branch4/LConn1 -- "Bus 5 "/RConn1 -- Three-Phase Series RLC Branch1/RConn1 -- Three-Phase Series RLC Branch20/RConn1 -- Three-Phase Series RLC Branch7/RConn1
  Three-Phase Series RLC Branch7/RConn3 -- "Bus 5 "/RConn3 -- Three-Phase Series RLC Branch1/RConn3 -- Three-Phase Series RLC Branch4/LConn3 -- Three-Phase Series RLC Branch20/RConn3
  Three-Phase Series RLC Branch15/RConn2 -- "Bus 12 "/LConn2 -- Three-Phase Series RLC Branch13/RConn2
  Three-Phase Series RLC Branch19/LConn1 -- "Bus 10 "/LConn1 -- Three-Phase Series RLC Branch17/LConn1
  Three-Phase Transformer (Two Windings)3/RConn1 -- "Bus 6 "/LConn1 -- Three-Phase Series RLC Load4/LConn1
  Three-Phase Series RLC Branch4/RConn2 -- "Bus 6 "/RConn2 -- Three-Phase Series RLC Branch15/LConn2 -- Three-Phase Series RLC Branch18/LConn2 -- Three-Phase Series RLC Branch12/LConn2
  Three-Phase Series RLC Branch14/LConn3 -- "Bus 14 "/LConn3 -- Three-Phase Series RLC Branch16/LConn3
  Three-Phase Series RLC Branch18/RConn3 -- "Bus 11 "/LConn3 -- Three-Phase Series RLC Branch19/RConn3
  Three-Phase Series RLC Branch7/RConn2 -- "Bus 5 "/RConn2 -- Three-Phase Series RLC Branch1/RConn2 -- Three-Phase Series RLC Branch4/LConn2 -- Three-Phase Series RLC Branch20/RConn2
  Three-Phase Transformer (Two Windings)1/RConn1 -- "Bus 2 "/LConn1 -- Three-Phase Series RLC Load11/LConn1
  Three-Phase Series RLC Branch8/RConn2 -- Three-Phase Series RLC Branch10/LConn2 -- "Bus 4 "/RConn2 -- Three-Phase Series RLC Branch1/LConn2 -- Three-Phase Series RLC Branch5/RConn2 -- Three-Phase Series RLC Branch6/RConn2
  "Bus 3 "/LConn3 -- Three-Phase Series RLC Load12/LConn3 -- Three-Phase Transformer (Two Windings)2/RConn3
  Three-Phase Series RLC Branch19/LConn2 -- "Bus 10 "/LConn2 -- Three-Phase Series RLC Branch17/LConn2
  Three-Phase Series RLC Branch9/RConn3 -- "Bus 7 "/RConn3 -- Three-Phase Series RLC Branch10/RConn3
  "Bus 3 "/LConn1 -- Three-Phase Series RLC Load12/LConn1 -- Three-Phase Transformer (Two Windings)2/RConn1
  Three-Phase Series RLC Branch4/RConn1 -- "Bus 6 "/RConn1 -- Three-Phase Series RLC Branch12/LConn1 -- Three-Phase Series RLC Branch18/LConn1 -- Three-Phase Series RLC Branch15/LConn1
  Three-Phase Series RLC Branch18/LConn3 -- "Bus 6 "/RConn3 -- Three-Phase Series RLC Branch4/RConn3 -- Three-Phase Series RLC Branch15/LConn3 -- Three-Phase Series RLC Branch12/LConn3
  Three-Phase Series RLC Branch3/RConn3 -- "Bus 3 "/RConn3 -- Three-Phase Series RLC Branch5/LConn3
  Three-Phase Series RLC Branch3/LConn2 -- "Bus 2 "/RConn2 -- Three-Phase Series RLC Branch20/LConn2 -- Three-Phase Series RLC Branch6/LConn2 -- Three-Phase Series RLC Branch2/RConn2
  Three-Phase Series RLC Branch8/LConn1 -- "Bus 9 "/LConn1 -- Three-Phase Series RLC Branch16/RConn1 -- Three-Phase Series RLC Branch17/RConn1 -- Three-Phase Series RLC Branch11/RConn1
  Three-Phase Series RLC Branch8/LConn3 -- Three-Phase Series RLC Branch11/RConn3 -- "Bus 9 "/LConn3 -- Three-Phase Series RLC Branch16/RConn3 -- Three-Phase Series RLC Branch17/RConn3
  Three-Phase Series RLC Branch18/RConn2 -- "Bus 11 "/LConn2 -- Three-Phase Series RLC Branch19/RConn2
  Three-Phase Series RLC Branch12/RConn3 -- "Bus 13 "/LConn3 -- Three-Phase Series RLC Branch14/RConn3 -- Three-Phase Series RLC Branch13/LConn3
  Three-Phase Transformer (Two Windings)1/RConn3 -- "Bus 2 "/LConn3 -- Three-Phase Series RLC Load11/LConn3
  Three-Phase Transformer (Two Windings)4/LConn1 -- "Bus 8 "/RConn1
  "Bus 7 "/LConn3 -- Three-Phase Series RLC Branch11/LConn3
  Three-Phase Series RLC Load8/LConn2 -- "Bus 12 "/RConn2
  Three-Phase Series RLC Branch11/LConn2 -- "Bus 7 "/LConn2
  Synchronous Compensator/RConn2 -- Three-Phase Transformer (Two Windings)4/RConn2
  Three-Phase V-I Measurement/RConn3 -- Three-Phase Transformer (Two Windings)5/RConn3
  Three-Phase V-I Measurement1/LConn2 -- "Bus 5 "/LConn2
  " Generator1"/RConn1 -- Three-Phase Transformer (Two Windings)5/LConn1
  "Bus 8 "/RConn3 -- Three-Phase Transformer (Two Windings)4/LConn3
  " Generator"/RConn2 -- Three-Phase Transformer (Two Windings)1/LConn2
  " Generator"/RConn3 -- Three-Phase Transformer (Two Windings)1/LConn3
  Three-Phase Series RLC Load7/LConn3 -- "Bus 11 "/RConn3
  Three-Phase Series RLC Load5/LConn2 -- Three-Phase V-I Measurement2/LConn2
  Synchronous Compensator/RConn3 -- Three-Phase Transformer (Two Windings)2/LConn3
  "Bus 14 "/RConn2 -- Three-Phase V-I Measurement3/RConn2
  Three-Phase V-I Measurement/LConn3 -- "Bus 1 "/LConn3
  Synchronous Compensator/RConn2 -- Three-Phase Transformer (Two Windings)2/LConn2
  "Synchronous Compensator "/RConn1 -- Three-Phase Transformer (Two Windings)3/LConn1
  Three-Phase Series RLC Branch11/LConn1 -- "Bus 7 "/LConn1
  "Synchronous Compensator "/RConn2 -- Three-Phase Transformer (Two Windings)3/LConn2
  Synchronous Compensator/RConn1 -- Three-Phase Transformer (Two Windings)4/RConn1
  "Bus 8 "/RConn2 -- Three-Phase Transformer (Two Windings)4/LConn2
  Current Measurement/LConn1 -- Three-Phase V-I Measurement3/LConn1
  "Bus 4 "/LConn2 -- Three-Phase Series RLC Load1/LConn2
  Current Measurement/RConn1 -- Three-Phase Series RLC Load10/LConn1
  "Bus 14 "/RConn3 -- Three-Phase V-I Measurement3/RConn3
  Three-Phase Series RLC Load9/LConn3 -- "Bus 13 "/RConn3
  Three-Phase V-I Measurement/LConn2 -- "Bus 1 "/LConn2
  "Bus 4 "/LConn3 -- Three-Phase Series RLC Load1/LConn3
  Three-Phase Series RLC Load9/LConn1 -- "Bus 13 "/RConn1
  Three-Phase Series RLC Load8/LConn1 -- "Bus 12 "/RConn1
  Three-Phase Series RLC Branch9/LConn1 -- "Bus 8 "/LConn1
  Synchronous Compensator/RConn1 -- Three-Phase Transformer (Two Windings)2/LConn1
  Current Measurement1/RConn1 -- Three-Phase Series RLC Load10/LConn2
  Current Measurement1/LConn1 -- Three-Phase V-I Measurement3/LConn2
  Three-Phase Series RLC Load6/LConn3 -- "Bus 10 "/RConn3
  Three-Phase Series RLC Load5/LConn1 -- Three-Phase V-I Measurement2/LConn1
  Current Measurement2/RConn1 -- Three-Phase Series RLC Load10/LConn3
  Three-Phase Series RLC Load9/LConn2 -- "Bus 13 "/RConn2
  " Generator"/RConn1 -- Three-Phase Transformer (Two Windings)1/LConn1
  Three-Phase Series RLC Load8/LConn3 -- "Bus 12 "/RConn3
  Three-Phase V-I Measurement/RConn2 -- Three-Phase Transformer (Two Windings)5/RConn2
  "Bus 4 "/LConn1 -- Three-Phase Series RLC Load1/LConn1
  Three-Phase V-I Measurement2/RConn2 -- "Bus 9 "/RConn2
  Three-Phase V-I Measurement1/LConn1 -- "Bus 5 "/LConn1
  " Generator1"/RConn2 -- Three-Phase Transformer (Two Windings)5/LConn2
  Three-Phase V-I Measurement1/RConn1 -- Three-Phase Series RLC Load3/LConn1
  Three-Phase V-I Measurement1/RConn2 -- Three-Phase Series RLC Load3/LConn2
  Three-Phase V-I Measurement1/LConn3 -- "Bus 5 "/LConn3
  Three-Phase V-I Measurement2/RConn1 -- "Bus 9 "/RConn1
  Three-Phase Series RLC Load5/LConn3 -- Three-Phase V-I Measurement2/LConn3
  Three-Phase V-I Measurement/LConn1 -- "Bus 1 "/LConn1
  Synchronous Compensator/RConn3 -- Three-Phase Transformer (Two Windings)4/RConn3
  Three-Phase V-I Measurement/RConn1 -- Three-Phase Transformer (Two Windings)5/RConn1
  Three-Phase Series RLC Load6/LConn2 -- "Bus 10 "/RConn2
  Three-Phase V-I Measurement2/RConn3 -- "Bus 9 "/RConn3
  "Synchronous Compensator "/RConn3 -- Three-Phase Transformer (Two Windings)3/LConn3
  Three-Phase Series RLC Branch9/LConn2 -- "Bus 8 "/LConn2
  "Bus 14 "/RConn1 -- Three-Phase V-I Measurement3/RConn1
  "Bus 11 "/RConn1 -- Three-Phase Series RLC Load7/LConn1
  Current Measurement2/LConn1 -- Three-Phase V-I Measurement3/LConn3
  Three-Phase Series RLC Load6/LConn1 -- "Bus 10 "/RConn1
  "Bus 11 "/RConn2 -- Three-Phase Series RLC Load7/LConn2
  Three-Phase V-I Measurement1/RConn3 -- Three-Phase Series RLC Load3/LConn3
  Three-Phase Series RLC Branch9/LConn3 -- "Bus 8 "/LConn3
  " Generator1"/RConn3 -- Three-Phase Transformer (Two Windings)5/LConn3
